simulink model "turbo_controller"  (R2025a)
settings: Solver=FixedStepAuto  StartTime=0.0  StopTime=inf  FixedStep=0.001  RelTol=1e-3
PostLoadFcn:
  | % 自动定位同目录CubeMX文件；不需要外部初始化脚本。
  | codertarget.data.setParameterValue('turbo_controller','STM32CubeMX.ProjectFile',fullfile(fileparts(get_param('turbo_controller','FileName')),'turbo_f407.ioc'));
InitFcn:
  | % 中文说明：按原控制器字段与类型创建三组接口总线；控制参数已内嵌。
  | tc_names=["EValve_Cycle" "EValve_Open" "Eblast_Cycle" "Eblast_Open" "Motor_Cycle" "Motor_Open" "EValve_Enable" "Eblast_Enable" "Motor_Enable" "SWO_Firework" "SWO_BleedAir" "EngineState" "Flag_ECUReset_Clear" "Flag_ECUReset_Save" "Flag_Reset_Enable" "Accelerator" "Nc_dem" "Nc"]; tc_types=["uint16" "uint16" "uint16" "uint16" "uint16" "uint16" "uint8" "uint8" "uint8" "uint8" "uint8" "uint8" "uint8" "uint8" "uint8" "single" "single" "single"];
  | for tc_k=1:numel(tc_names)
  |  tc_e(tc_k)=Simulink.BusElement; tc_e(tc_k).Name=char(tc_names(tc_k)); tc_e(tc_k).DataType=char(tc_types(tc_k));
  | end
  | EngineControl_Out=Simulink.Bus; EngineControl_Out.DataScope='Exported'; EngineControl_Out.Elements=tc_e;
  | clear tc_e tc_names tc_types tc_k
  | tc_names=["savedata1" "savedata2" "savedata3" "savedata4" "savedata5" "savedata6" "savedata7" "savedata8" "savedata9" "savedata10" "savedata11" "savedata12" "savedata13" "savedata14" "savedata15" "savedata16" "savedata17" "savedata18" "savedata19" "savedata20" "savedata21" "savedata22" "savedata23" "savedata24" "savedata25"]; tc_types=["single" "single" "single" "single" "single" "single" "single" "single" "single" "single" "single" "single" "single" "single" "single" "single" "single" "single" "single" "single" "single" "single" "single" "single" "single"];
  | for tc_k=1:numel(tc_names)
  |  tc_e(tc_k)=Simulink.BusElement; tc_e(tc_k).Name=char(tc_names(tc_k)); tc_e(tc_k).DataType=char(tc_types(tc_k));
  | end
  | SaveData_Out=Simulink.Bus; SaveData_Out.DataScope='Exported'; SaveData_Out.Elements=tc_e;
  | clear tc_e tc_names tc_types tc_k
  | tc_names=["senddata1" "senddata2" "senddata3" "senddata4" "senddata5" "senddata6" "senddata7" "senddata8" "senddata9" "senddata10" "senddata11" "senddata12" "senddata13" "senddata14" "senddata15" "senddata16" "senddata17" "senddata18" "senddata19" "senddata20" "senddata21" "senddata22" "senddata23" "senddata24" "senddata25" "senddata26" "senddata27" "senddata28" "senddata29"]; tc_types=["uint8" "uint8" "uint8" "uint8" "uint8" "uint8" "uint8" "uint8" "uint8" "uint8" "uint8" "uint8" "uint8" "uint8" "uint8" "uint8" "uint8" "uint8" "uint8" "uint8" "uint8" "uint8" "uint8" "uint8" "uint8" "uint8" "uint8" "uint8" "uint8"];
  | for tc_k=1:numel(tc_names)
  |  tc_e(tc_k)=Simulink.BusElement; tc_e(tc_k).Name=char(tc_names(tc_k)); tc_e(tc_k).DataType=char(tc_types(tc_k));
  | end
  | SendData_Out=Simulink.Bus; SendData_Out.DataScope='Exported'; SendData_Out.Elements=tc_e;
  | clear tc_e tc_names tc_types tc_k
  | 
  | % 以下为接口中文说明；只设置描述，不改变数值或数据类型。
  | EngineControl_Out.Description='执行控制输出（阀、电机、点火、状态及复位请求）';
  | tc_cn=["EValve_Cycle（主油阀周期计数（每计数2毫秒））" "EValve_Open（主油阀开通计数（每计数2毫秒））" "Eblast_Cycle（副油阀周期计数（每计数2毫秒））" "Eblast_Open（副油阀开通计数（每计数2毫秒））" "Motor_Cycle（起动电机周期计数）" "Motor_Open（起动电机开通计数）" "EValve_Enable（主油阀驱动使能）" "Eblast_Enable（副油阀驱动使能）" "Motor_Enable（起动电机使能）" "SWO_Firework（点火器使能（1开））" "SWO_BleedAir（引气阀使能（1开））" "EngineState（发动机状态）" "Flag_ECUReset_Clear（清除复位恢复状态请求）" "Flag_ECUReset_Save（保存复位恢复数据请求）" "Flag_Reset_Enable（处理器软件复位请求）" "Accelerator（油门／油泵给定控制量）" "Nc_dem（控制目标转速）" "Nc（发动机反馈转速（转每分））"];
  | tc_elements=EngineControl_Out.Elements;
  | for tc_k=1:numel(tc_cn)
  |  tc_elements(tc_k).Description=char(tc_cn(tc_k));
  | end
  | EngineControl_Out.Elements=tc_elements;
  | clear tc_cn tc_elements tc_k
  | SaveData_Out.Description='25项运行记录；字段含义按当前模型数据来源解释';
  | tc_cn=["savedata1（指令回显记录）" "savedata2（入口总温记录（℃））" "savedata3（电源电压记录）" "savedata4（排气温度记录（℃））" "savedata5（标定燃油压力记录）" "savedata6（副油阀占空比记录（％））" "savedata7（主油阀占空比记录（％））" "savedata8（温度修正转速记录）" "savedata9（开关输出及反馈位域）" "savedata10（物理转速记录）" "savedata11（油泵目标给定原始值）" "savedata12（起动电机占空比记录（％））" "savedata13（发动机状态码记录）" "savedata14（故障告警位域记录）" "savedata15（模型记录帧序号）" "savedata16（处理器温度记录（℃））" "savedata17（装订转速记录（沿用旧电源字段名））" "savedata18（导航高度记录）" "savedata19（飞行空速记录）" "savedata20（主阀旧记录位（恒零保留））" "savedata21（第21项保留记录（恒零））" "savedata22（保留记录项22）" "savedata23（保留记录项23）" "savedata24（保留记录项24）" "savedata25（保留记录项25）"];
  | tc_elements=SaveData_Out.Elements;
  | for tc_k=1:numel(tc_cn)
  |  tc_elements(tc_k).Description=char(tc_cn(tc_k));
  | end
  | SaveData_Out.Elements=tc_elements;
  | clear tc_cn tc_elements tc_k
  | SendData_Out.Description='29字段回传及外设命令接口；板端上位机帧只取第3至27字段';
  | tc_cn=["senddata1（回传发送允许标志（不直接上线路））" "senddata2（回传载荷长度25字节）" "senddata3（回传指令回显字节）" "senddata4（总温编码字节（℃＋80））" "senddata5（电源电压编码字节）" "senddata6（排温编码高字节）" "senddata7（排温编码低字节）" "senddata8（燃油压力编码高字节）" "senddata9（燃油压力编码低字节）" "senddata10（副油阀占空比字节（％））" "senddata11（主油阀占空比字节（％））" "senddata12（修正转速编码高字节）" "senddata13（修正转速编码低字节）" "senddata14（驱动及反馈状态位域）" "senddata15（物理转速编码高字节）" "senddata16（物理转速编码低字节）" "senddata17（油泵目标给定高字节（串口二使用））" "senddata18（油泵目标给定低字节（串口二使用））" "senddata19（起动电机占空比命令（串口一使用））" "senddata20（发动机状态码字节）" "senddata21（故障告警位域字节）" "senddata22（帧序号占位（板端另行填写））" "senddata23（处理器温度编码（℃＋50））" "senddata24（控制目标转速编码高字节）" "senddata25（控制目标转速编码低字节）" "senddata26（占位字节（板端改填实测泵速高字节））" "senddata27（占位字节（板端改填实测泵速低字节））" "senddata28（装订转速高字节（本板未发送））" "senddata29（装订转速低字节（本板未发送））"];
  | tc_elements=SendData_Out.Elements;
  | for tc_k=1:numel(tc_cn)
  |  tc_elements(tc_k).Description=char(tc_cn(tc_k));
  | end
  | SendData_Out.Elements=tc_elements;
  | clear tc_cn tc_elements tc_k
  | 
  | 
  | % FRAM模块化事务：接口类型和上电初始状态，随模型保存，无外部初始化文件。
  | clear FM_elements
  | FM_elements(1)=Simulink.BusElement;FM_elements(1).Name='phase';FM_elements(1).DataType='uint8';FM_elements(1).Dimensions=[1 1];FM_elements(1).Description='phase（当前事务阶段）';
  | FM_elements(2)=Simulink.BusElement;FM_elements(2).Name='a';FM_elements(2).DataType='uint8';FM_elements(2).Dimensions=[64 1];FM_elements(2).Description='a（启动时缓存的首区64字节）';
  | FM_elements(3)=Simulink.BusElement;FM_elements(3).Name='active';FM_elements(3).DataType='uint16';FM_elements(3).Dimensions=[1 1];FM_elements(3).Description='active（当前有效记录区地址）';
  | FM_elements(4)=Simulink.BusElement;FM_elements(4).Name='generation';FM_elements(4).DataType='uint32';FM_elements(4).Dimensions=[1 1];FM_elements(4).Description='generation（当前有效记录代号）';
  | FM_elements(5)=Simulink.BusElement;FM_elements(5).Name='record';FM_elements(5).DataType='uint8';FM_elements(5).Dimensions=[64 1];FM_elements(5).Description='record（本次冻结的待写记录）';
  | FM_elements(6)=Simulink.BusElement;FM_elements(6).Name='addr';FM_elements(6).DataType='uint16';FM_elements(6).Dimensions=[1 1];FM_elements(6).Description='addr（本次备用写入地址）';
  | FM_elements(7)=Simulink.BusElement;FM_elements(7).Name='lastSave';FM_elements(7).DataType='single';FM_elements(7).Dimensions=[1 1];FM_elements(7).Description='lastSave（上次开始保存的秒数）';
  | FM_elements(8)=Simulink.BusElement;FM_elements(8).Name='lastState';FM_elements(8).DataType='uint8';FM_elements(8).Dimensions=[1 1];FM_elements(8).Description='lastState（上次保存时的发动机状态）';
  | FM_elements(9)=Simulink.BusElement;FM_elements(9).Name='boot';FM_elements(9).DataType='boolean';FM_elements(9).Dimensions=[1 1];FM_elements(9).Description='boot（启动记录是否允许恢复）';
  | FM_elements(10)=Simulink.BusElement;FM_elements(10).Name='consumed';FM_elements(10).DataType='boolean';FM_elements(10).Dimensions=[1 1];FM_elements(10).Description='consumed（本次启动恢复通知是否已发送）';
  | FM_elements(11)=Simulink.BusElement;FM_elements(11).Name='payload';FM_elements(11).DataType='uint8';FM_elements(11).Dimensions=[20 1];FM_elements(11).Description='payload（当前20字节恢复内容）';
  | ... (+35 lines)
model workspace (MAT data in the model file):
  CRC16_Table_Reference = [0 4129 8258 12387 16516 20645 24774 28903 33032 37161 41290 45419 ... (256 elements, 256x1)]
  PE_Kaer = [0.15402 0.15402 0.12264 0.10076 0.09481 0.07601 0.07111 0.0569 0.05198 0.04926 0.05308 0.04325 ... (13 elements, 1x13)]
  PE_Nr = [21.2982 61.4260372 67.7475458 72.7394382 76.845934 80.6988798 83.8449282 86.6491912 88.9382406 89.178606 91.1938214 93.4068058 ... (13 elements, 1x13)]
  PE_Pump_Translate = 33.5999984741
  PE_RotaSpeed_Translate = 860
  PE_Taer = [0.4939154 0.4939154 0.40780982 0.34066978 0.31622756 0.30405716 0.34300244 0.26785022 0.37393554 0.23914836 0.44563948 0.31044662 ... (13 elements, 1x13)]
  PF_ACCFULLRANGE = 3360
  PF_Flag_ECUReset = 0
  PF_Flag_rx_suc = 1
  PF_Gear_Info = [40000; 45000; 50000; 55000; 57000; 59000; 60000; 61000; 61000; 61000; 61000; 61000]
  PF_K_TiaoJie = 1
  PF_Kpu = 10
  PF_MySet_Rxdata = [0 0 0 0 0 0 0 0 0 0 0 0 ... (50 elements, 50x1)]
  PF_MyUsart1_Rxdata = [0 0 0 0 0 0 0 0 0 0 0 0 ... (50 elements, 50x1)]
  PF_MyUsart2_Rxdata = [0 0 0 0 0 0 0 0 0 0 0 0 ... (50 elements, 50x1)]
  PF_Reset_Information = [0 0 0 0 0 0 0 0 0 0 0 0 ... (20 elements, 20x1)]
  PF_Sensor_X1_T4 = [0 4095]
  PF_Sensor_X2_T4 = [0 1.66666698456]
  PF_Sensor_X3_T4 = [0 504 999 1497 2010 2529 3051 3568 4076 4571 4959]
  PF_Sensor_X_P2 = [0.5 3]
  PF_Sensor_X_Poil = [0.5 3]
  PF_Sensor_X_T1t = [-50 300]
  PF_Sensor_X_Vpower = [0 3]
  PF_Sensor_X_Vpump = [0 3]
  PF_Sensor_Y1_T4 = [0 3]
  PF_Sensor_Y2_T4 = [0 5000]
  PF_Sensor_Y3_T4 = [0 100 200 300 400 500 600 700 800 900 980]
  PF_Sensor_Y_P2 = [0 1000]
  PF_Sensor_Y_Poil = [0 1000]
  PF_Sensor_Y_T1t = [-50 300]
  PF_Sensor_Y_Vpower = [0 33]
  PF_Sensor_Y_Vpump = [0 33]
  PG_CtrlMode_CloseLoop : mpt.Parameter (value not decoded)
  PG_CtrlMode_ManualAcc : mpt.Parameter (value not decoded)
  PG_CtrlMode_Origin : mpt.Parameter (value not decoded)
  PG_CtrlMode_Start : mpt.Parameter (value not decoded)
  PG_CtrlMode_Stop : mpt.Parameter (value not decoded)
  PG_ES_Clp : mpt.Parameter (value not decoded)
  PG_ES_EngStart : mpt.Parameter (value not decoded)
  PG_ES_Manual : mpt.Parameter (value not decoded)
  PG_ES_Origin : mpt.Parameter (value not decoded)
  PG_ES_Stop : mpt.Parameter (value not decoded)
  PG_Instr_BleedAirSet : mpt.Parameter (value not decoded)
  PG_Instr_CloseLoop : mpt.Parameter (value not decoded)
  PG_Instr_ECUReSet : mpt.Parameter (value not decoded)
  PG_Instr_EValveSet : mpt.Parameter (value not decoded)
  PG_Instr_EblastSet : mpt.Parameter (value not decoded)
  PG_Instr_Erase : mpt.Parameter (value not decoded)
  PG_Instr_FireWorkSet : mpt.Parameter (value not decoded)
  PG_Instr_ManualPlus : mpt.Parameter (value not decoded)
  PG_Instr_ManualrReduce : mpt.Parameter (value not decoded)
  PG_Instr_MotorSet : mpt.Parameter (value not decoded)
  PG_Instr_OilSet : mpt.Parameter (value not decoded)
  PG_Instr_SelfCheck : mpt.Parameter (value not decoded)
  PG_Instr_Start : mpt.Parameter (value not decoded)
  PG_Instr_Stop : mpt.Parameter (value not decoded)
  PG_Instr_StopZero : Simulink.Parameter (value not decoded)
  PG_Location_Air : Simulink.Parameter (value not decoded)
  PG_Location_Gnd : Simulink.Parameter (value not decoded)
  PG_ServoCtrlMode_CloseLoop : Simulink.Parameter (value not decoded)
  PG_ServoCtrlMode_CloseLoopMax : Simulink.Parameter (value not decoded)
  PG_ServoCtrlMode_CloseLoopMin : Simulink.Parameter (value not decoded)
  PG_ServoCtrlMode_ManualAcc : Simulink.Parameter (value not decoded)
  PG_ServoCtrlMode_ManualAccMax : Simulink.Parameter (value not decoded)
  PG_ServoCtrlMode_ManualAccMin : Simulink.Parameter (value not decoded)
  PG_SpeedDot_Permit : Simulink.Parameter (value not decoded)
  PL_EngineModel_Actuator = [0 10 100]
  PL_EngineModel_EngineStar_Press_P2 = [1013 1098.4 1099.144828 1099.931034 1103.613793 1162.662069 1143.793103 1131.006897 1123.186207 1117.6 1114 1111.806897 ... (127 elements, 1x127)]
  PL_EngineModel_EngineStar_RotaSpeed = [200 2000 9584 9660 10220 10240 10260 10288 10308 10368 10380 10408 ... (127 elements, 1x127)]
  PL_EngineModel_EngineStar_Temp_Exhaust = [128 129 129.1 130 131 131.1 132 133 134 134.1 135 135.1 ... (127 elements, 1x127)]
  PL_EngineModel_EngineStar_Time = [0.05 0.1 0.15 0.2 0.25 0.3 0.35 0.4 0.45 0.5 0.55 0.6 ... (127 elements, 1x127)]
  PL_EngineModel_IdleAbove_Nr = [0 21.2982 61.4260372 67.7475458 72.7394382 76.845934 80.6988798 83.8449282 86.6491912 88.9382406 89.178606 91.1938214 ... (14 elements, 1x14)]
  PL_EngineModel_IdleAbove_P2r = [0.986923266716 1.57907722675 1.81593881076 1.99358499877 2.23044658278 2.43770046879 2.65482358747 2.84233900814 3.03972366149 3.18776215149 3.25684678016 3.3950160375 ... (14 elements, 1x14)]
  PL_EngineModel_IdleAbove_Tempr = [0.0536001429337 1.07200285867 1.63301768805 1.63659103091 1.66875111667 1.72592460247 1.77595140254 1.86171163123 1.95461854565 2.03323208862 2.03323208862 2.13685903162 ... (14 elements, 1x14)]
  PL_EngineModel_IdleAbove_Ter = [0.42434128 0.42434128 0.42434128 0.30669408 0.23570008 0.22150128 0.1997974 0.23803274 0.16115638 0.24279948 0.13600422 0.31308354 ... (14 elements, 1x14)]
  PL_EngineModel_IdleAbove_Wfr = [0 10.142 23.8337 27.8905 31.9473 36.0041 40.0609 44.1177 48.1745 52.2313 52.7384 56.7952 ... (14 elements, 1x14)]
  PL_EngineModel_Press_P2 = [400 400 400 400 400 400 400 400 400 400]
  PL_EngineModel_Rotaspeed = [0 20000 96400]
  PL_EngineModel_Temp_Exhaust = [500 500 500 500 500 500 500 500 500 500]
  PL_Kaer = [0.1 0.1 0.1 0.1 0.1 0.1]
  PL_Nr = [50 60 70 80 90 100]
  PL_Taer = [0.1 0.1 0.1 0.1 0.1 0.1]
  Sig : Simulink.Signal (value not decoded)
  Ts_ms : Simulink.Parameter (value not decoded)
  false : Simulink.Parameter (value not decoded)
  true : Simulink.Parameter (value not decoded)
symbols that are objects in the model workspace (value not decoded): PG_CtrlMode_CloseLoop, PG_CtrlMode_ManualAcc, PG_CtrlMode_Origin, PG_CtrlMode_Start, PG_CtrlMode_Stop, PG_ES_Clp, PG_ES_EngStart, PG_ES_Manual, PG_ES_Origin, PG_ES_Stop, PG_Instr_BleedAirSet, PG_Instr_CloseLoop, PG_Instr_EblastSet, PG_Instr_ECUReSet, PG_Instr_Erase, PG_Instr_EValveSet, PG_Instr_FireWorkSet, PG_Instr_ManualPlus, PG_Instr_ManualrReduce, PG_Instr_MotorSet, PG_Instr_OilSet, PG_Instr_SelfCheck, PG_Instr_Start, PG_Instr_Stop, PG_Instr_StopZero, PG_ServoCtrlMode_CloseLoop, PG_ServoCtrlMode_CloseLoopMax, PG_ServoCtrlMode_CloseLoopMin, PG_ServoCtrlMode_ManualAcc, PG_ServoCtrlMode_ManualAccMax, PG_ServoCtrlMode_ManualAccMin, Ts_ms
libraries: simulink x97, stm32blockslib x10, stm32f4xxblockslib x8
(part 7 of 26)

== system turbo_controller/BoardInput_输入换算与协议解析/In03_Pump（油泵回包预留校验） ==
  note: 输入侧油泵回包的预留检查
      |
      | 本模块接收油泵串口字节和有效数量，内部Receive按AA55帧头拼接22字节帧，再检查CRC16。分批到达
      | 的帧可以依靠缓存接着收，校验失败不会变成有效帧。
      |
      | 它保留的是输入侧原有预留校验路径，当前该结果没有用来更新控制转速或实际回传泵速。不要因为这
      | 里名为Pump，就把它当成最终泵速反馈来源。
      |
      | 实际用于上位机回传的油泵反馈，在BoardOutput/Out01_Pump中处理：同样检查22字节帧，提取第6、7
      | 字节并作0.875/0.125平滑。本模块没有取代那条路径，也不生成发往油泵的控制命令。
  Rx（串口接收字节）_237 : Inport  OutDataTypeStr=uint8
  Count（有效字节数）_238 : Inport  Port=2  OutDataTypeStr=uint32
  Format（保持原输出维度）_1 : Reshape
  Receive（逐字节组帧与保持有效结果）_353 : Subsystem  Description=|
      | 预留油泵校验接收流程：按1→2→3→4阅读
      | 
      | 第一步只遍历本批有效字节，最多处理64项；第二步识别AA55、收齐22字节，并保存尚未收完的半帧；第三步确认本字节刚收齐且CRC通过；第四步统计这一批是否出现过有效帧。
      | 
      | Loop在一次调用内逐字节重复这些步骤，不是每一步各等1 ms。接收数组的Index每批重新遍历，收帧Position可以跨批保留，两者不是同一个位置。
      | 
      | 本分支输出本批是否出现有效帧，不生成实际平滑泵速。实际泵速来自BoardOutput/Out01_Pump的接收路径。
      | 
      | 本次将原有处理块按职责封装，保留原协议、初始化、数据类型、校验和循环行为。各步骤内部可看输入、公式和例子。
  Valid（原预留校验结果）_354 : Outport
  wires:
  Rx（串口接收字节）_237/1 -> Receive（逐字节组帧与保持有效结果）_353/1(Rx（本次接收字节）_239)  "Rx（串口接收字节）"
  Count（有效字节数）_238/1 -> Receive（逐字节组帧与保持有效结果）_353/2(Count（本次有效字节数）_240)  "Count（有效字节数）"
  Receive（逐字节组帧与保持有效结果）_353/1(Valid（原预留校验结果）_352) -> Format（保持原输出维度）_1/1  "Receive（逐字节组帧与保持有效结果）"
  Format（保持原输出维度）_1/1 -> Valid（原预留校验结果）_354/1

== system turbo_controller/BoardInput_输入换算与协议解析/In04_Capture（捕获间隔缓存） ==
  note: 捕获间隔缓存：把脉冲发生时刻整理成最近十个时间间隔
      |
      | 输入Capture是TIM3本批捕获读数，最多16项；输入Count只说明本批有几项新读数，Seconds为本次处
      | 理时刻，单位秒。当前定时器每增加1计数相当于1微秒。
      |
      | 按四块阅读：
      | Step01逐项取出本批有效捕获，超过本批数量或第16项就结束循环；
      | Step02保存上次捕获、十项间隔、写入位置、累计有效数和最近有效时间；
      | Step03根据本项捕获计算间隔，决定是否更新缓存和状态；
      | Step04只整理三个输出的维度，送后续测速。
      |
      | Step02与Step03之间是状态反馈，不是先等一个额外毫秒再处理。Loop会在同一次调用内遍历本批多个
      | 捕获；一个批次的末项读数也会留作下一批首项的差分基准。
      |
      | 输出Periods为最近十个间隔，Count为缓存里真正有效的间隔个数，LastTime为最近接受正间隔的处理
      | 时刻。输出Count与输入Count不是同一个数量。这里不直接输出转速；去极值与每转3脉冲换算在In05_
      | Speed/CaptureSpeed完成。
  Capture（最多十六个捕获计数）_355 : Inport  OutDataTypeStr=uint16
  Count（本次有效个数）_356 : Inport  Port=2  OutDataTypeStr=uint32
  Seconds（当前秒数）_357 : Inport  Port=3  OutDataTypeStr=double
  Loop（逐项处理循环）_358 : ForIterator  IterationLimit=16  ExternalIncrement=on  IterationVariableDataType=uint32
  Step01_逐项取出本批有效捕获 : Subsystem  Description=|
      | 第一步：按顺序取出本批捕获，不处理数组尾部旧值
      | 
      | 外层Loop给出从1开始的序号i。本项捕获=Capture(i)，本项有效=(i≤本批Count)。
      | 
      | 如果i已达到本批Count，或i=16，就把下一循环序号设17，结束循环；否则下一序号=i+1。因此输入数组虽然有16项，Count=3时只会把前3项当新捕获。Count=0时保留一次无效项处理，状态由后面保持，不写入新间隔。
      | 
      | 例：一批有[1000,2000,3000]三项，依次交给更新步骤处理；它们是在本次调用内顺序处理，不是分三毫秒执行。
      | 
      | 输出分别为本项捕获、有效许可和下一循环序号。i是本批数组位置，不是十项环形缓存的写入位置。
  Step02_保存捕获与缓存历史状态 : Subsystem  Description=|
      | 第二步：保留下一项计算还要用到的五种历史状态
      | 
      | 这里的五条记忆各有用途：
      | Previous：上一项有效捕获读数，用来求下一次差分，初值0；
      | Ring：最近十个已接受间隔，初值为十个0；
      | Index：下一次覆盖缓存的哪一项，初值1；
      | Count：已保存多少个有效间隔，初值0，最多10；
      | LastTime：最近接受正间隔的处理时刻，初值-1秒。
      | 
      | 每次把Step03给出的新状态按原类型保存：Previous为uint32，Index和Count为uint8，Ring和LastTime为single；下一次循环/调用再提供给Step03。
      | 
      | 不要把Previous、Ring和LastTime混为一份数据。读数用于差分，间隔用于测速，时间用于判断新鲜程度。没有有效捕获时，上游选择器会把旧状态送回来，记忆继续保持。
  Step03_计算间隔并更新环形缓存 : Subsystem  Description=|
      | 对一项捕获完成回卷差分和缓存更新
      | 
      | 输入为上一捕获、旧十项缓存、旧写入位置、旧有效数、旧最近时间，以及本次Capture、Seconds和Active。
      | 
      | 六步各做一件事：算回卷后的间隔、判断能否接受、生成缓存候选值、计算下一写入位置、计算有效数量、最后按许可提交状态。
      | 
      | 关键规则有两条：只要Active为真就更新Previous；但只有Active为真且间隔>0，才更新Ring、Index、Count和LastTime。重复读数的零间隔不会增加记录，也不刷新最近有效时间。
      | 
      | 例：上次65530、这次4，间隔为10；若本项有效，就存10并更新状态。若本项无效，即使算出了10，也保留全部旧状态。输出回到In04的历史记忆供下一项使用，不是给硬件发送命令。
  Step04_整理间隔数量和时间输出 : Subsystem  Description=|
      | 第四步：整理三个对外输出的形状，不再次计算
      | 
      | 将Step03输出的十项Ring整理为原工程的一维向量接口；累计有效数量和最近有效时间按原来要求整理为标量形状。
      | 
      | 数值不变、单位不变，也不做新的滤波。Periods仍是计数间隔，当前配置下可按微秒解释；Count仍为0～10；LastTime仍为秒。
      | 
      | 例如Ring中一项1000经过此处还是1000，不会变成1000转/分。真正的转速换算在后面的CaptureSpeed，超时判断在Status；本块只保证连接双方看到的数组形状与修改前一致。
  Periods（最近十个有效间隔）_416 : Outport
  Count（有效间隔数）_417 : Outport  Port=2
  LastTime（最近有效脉冲秒数）_418 : Outport  Port=3
  wires:
  Step04_整理间隔数量和时间输出/3(输出3_Format（保持原输出维度）) -> LastTime（最近有效脉冲秒数）_418/1
  Step04_整理间隔数量和时间输出/2(输出2_Format（保持原输出维度）) -> Count（有效间隔数）_417/1
  Step04_整理间隔数量和时间输出/1(输出1_Vector1D（保持原一维向量接口）) -> Periods（最近十个有效间隔）_416/1
  Step01_逐项取出本批有效捕获/3(输出3_本项捕获有效) -> Step03_计算间隔并更新环形缓存/8(Active（本项捕获有效）_381)
  Step01_逐项取出本批有效捕获/2(输出2_本项捕获读数) -> Step03_计算间隔并更新环形缓存/6(Capture（当前捕获计数）_379)
  Step02_保存捕获与缓存历史状态/5(输出5_上次有效间隔时刻) -> Step03_计算间隔并更新环形缓存/5(LastTime（最近有效脉冲时间）_378)
  Step02_保存捕获与缓存历史状态/4(输出4_累计有效间隔数) -> Step03_计算间隔并更新环形缓存/4(Count（有效间隔个数）_377)
  Step02_保存捕获与缓存历史状态/3(输出3_当前环形写入位置) -> Step03_计算间隔并更新环形缓存/3(Index（下一写入位置）_376)
  Step02_保存捕获与缓存历史状态/2(输出2_旧十项间隔缓存) -> Step03_计算间隔并更新环形缓存/2(Ring（十项间隔缓存）_375)
  Step02_保存捕获与缓存历史状态/1(输出1_上一捕获读数) -> Step03_计算间隔并更新环形缓存/1(Previous（上次捕获计数）_374)
  Step01_逐项取出本批有效捕获/1(输出1_下一序号或退出值17) -> Loop（逐项处理循环）_358/1
  Step03_计算间隔并更新环形缓存/4(Count（更新后的有效个数）_411) -> Step04_整理间隔数量和时间输出/1(输入1_更新后的有效间隔数), Step02_保存捕获与缓存历史状态/5(输入5_更新后的有效间隔数)  "更新后的有效间隔数"
  Step03_计算间隔并更新环形缓存/3(Index（下次写入位置）_409) -> Step02_保存捕获与缓存历史状态/4(输入4_下一环形写入位置)  "下一环形写入位置"
  Step03_计算间隔并更新环形缓存/1(Previous（下次差分基准）_405) -> Step02_保存捕获与缓存历史状态/3(输入3_下一差分基准)  "下一差分基准"
  Step03_计算间隔并更新环形缓存/5(LastTime（最近有效脉冲时间）_414) -> Step02_保存捕获与缓存历史状态/2(输入2_最近有效间隔处理时刻), Step04_整理间隔数量和时间输出/2(输入2_最近有效间隔处理时刻)  "最近有效间隔处理时刻"
  Step03_计算间隔并更新环形缓存/2(Ring（更新后的间隔缓存）_407) -> Step04_整理间隔数量和时间输出/3(输入3_更新后的十项间隔), Step02_保存捕获与缓存历史状态/1(输入1_更新后的十项间隔)  "更新后的十项间隔"
  Capture（最多十六个捕获计数）_355/1 -> Step01_逐项取出本批有效捕获/3(输入3_本批最多16项捕获数组)  "本批最多16项捕获数组"
  Count（本次有效个数）_356/1 -> Step01_逐项取出本批有效捕获/2(输入2_本批有效捕获个数)  "本批有效捕获个数"
  Loop（逐项处理循环）_358/1 -> Step01_逐项取出本批有效捕获/1(输入1_本批当前处理序号)  "本批当前处理序号"
  Seconds（当前秒数）_357/1 -> Step03_计算间隔并更新环形缓存/7(Seconds（当前秒数）_380)  "Seconds（当前秒数）"

== system turbo_controller/BoardInput_输入换算与协议解析/In05_Speed（转速来源选择与滤波） ==
  note: 电机反馈与捕获估速怎样选成控制转速
      |
      | 这里有两种候选转速：电机串口反馈Motor，以及十项捕获间隔算出的Captured。输出Speed送根层Cont
      | rolRate，再到ISM作进一步异常判断和滤波。
      |
      | 先由Clock20ms产生每20 ms更新许可。CaptureSpeed从有效间隔中去掉一个最大和一个最小，估算转速
      | ，并给出分母有效标志。Status判断：上一电机给定是否非零、是否还在10次节拍等待中、脉冲是否超
      | 过0.1 s未更新、间隔是否至少3项。
      |
      | Select按顺序选择：电机给定非零时优先Motor，并把等待计数清零；退出电机后先保持旧Speed，等待
      | 10次20 ms节拍，约0.2 s后再尝试捕获估速。
      | 等待结束后，脉冲超时则给零；未超时且数量足够、分母有效才采用Captured，否则保持旧值。
      |
      | 非20 ms更新时刻，Speed和等待计数都保持。因此“父级每1 ms运行”并不是每1 ms都切换转速来源。
      | Held是上次控制转速，WaitCount是切换过程的记忆。
  Periods（最近十项捕获间隔）_1 : Inport  OutDataTypeStr=single
  Count（有效间隔数）_2 : Inport  Port=2  OutDataTypeStr=uint8
  LastTime（最近脉冲时间）_3 : Inport  Port=3  OutDataTypeStr=single
  PreviousMotor（上一电机给定）_4 : Inport  Port=4  OutDataTypeStr=uint16
  MotorSpeed（电机反馈转速）_5 : Inport  Port=5  OutDataTypeStr=single
  Seconds（当前秒数）_6 : Inport  Port=6  OutDataTypeStr=double
  CaptureSpeed（去极值估算转速）_19 : Subsystem  Description=|
      | 把最近脉冲间隔换算成转速：先筛数据，再去极值，最后计算
      | 
      | 输入Periods最多十项，Count=n说明前几项有效。四步分别是：排除空位、去掉一个最大值和一个最小值、检查分母并避免除零、按每转3脉冲换算RPM。
      | 
      | 去极值后的和S=有效间隔之和-最大有效间隔-最小有效间隔。
      | 转速=60000000×(n-2)/(3×S)，间隔采用微秒时，输出单位为转/分。
      | 
      | 例如十项都为1000微秒，去掉两项后S=8000，转速=60000000×8/(3×8000)=20000。去极值减轻单个偏大/偏小间隔的影响，不是无条件识别所有错误脉冲。
      | 
      | 本模块Valid只表示S>0。至少有3项的要求、最近脉冲是否超时、是否优先采用电机串口反馈，由外层Status和Select决定。数据不足时即使这里有一个数，也不能绕过这些条件直接用作控制反馈。
  Clock20ms（二十毫秒更新节拍）_18 : Subsystem  Description=|
      | 从秒数产生每二十毫秒一次的许可
      | 
      | 本模块收到当前模型时间Seconds。先乘1000换成毫秒，再对20取余，判断余数是否小于1：
      | 工作许可 = mod(Seconds×1000,20)<1。
      | 
      | 在父级1 ms离散调用下，约在0、20、40、60 ms等时刻为真，中间毫秒为假。用“小于1”表示当前1 ms时间格，避免把它理解成连续时间的一次精确相等判断。
      | 
      | 这只是一个布尔许可，不会让模型等待或暂停。转速选择用它决定何时更新Speed，回传组帧用它决定何时生成新帧；其他1 ms任务继续正常运行。
  Format（保持原输出维度）_1 : Reshape
  Held（保持的控制转速）_7 : UnitDelay  InitialCondition=single(0)  SampleTime=-1  HasFrameUpgradeWarning=on
  Select（优先级与保持选择）_65 : Subsystem  Description=|
      | 按优先级决定这一周期输出哪种转速
      | 
      | 输入包含20 ms许可、四个来源条件、捕获分母有效标志，两种候选转速，以及上次Speed和等待次数。处理顺序很重要。
      | 
      | 先看20 ms许可：本毫秒不到更新时间，就保持上次Speed和等待次数。
      | 到更新时间后，如果UseMotor成立，直接采用电机反馈Motor，同时等待次数清零。
      | 如果不再使用Motor，但Waiting仍成立，则保持旧Speed，并将等待次数加1，最多等待10次节拍。
      | 
      | 等待结束后，先看捕获是否Timeout：超时就输出0。未超时时，Enough和Valid同时成立才采用Captured；数量不够或分母无效时仍保持Held。
      | 
      | 例如电机刚停止给定，不会立刻切到可能还未准备好的捕获值，而先保持约0.2 s。Speed和WaitCount输出在父级被保存，下一次再作为历史输入，所以不能删除这两条记忆反馈。
  Status（来源与超时判定）_39 : Subsystem  Description=|
      | 转速来源现在是否可用
      | 
      | 这里不计算转速，而把输入整理成四个供Select使用的布尔条件。
      | 
      | UseMotor：上一周期电机给定大于0，表示电机仍在被驱动，优先采用电机串口反馈。
      | Waiting：等待次数小于10，表示从电机反馈退出后还在过渡期。等待次数由外层按20 ms节拍推进，10次约0.2 s。
      | Timeout：当前秒数减最近有效脉冲时间大于0.1 s，表示捕获结果已经不够新鲜。
      | Enough：有效间隔数至少3，保证去掉最大和最小之后还有数据。
      | 
      | 例如已有10项间隔，但最后一次脉冲是0.3 s前，Enough虽为真，Timeout也为真，仍不能把旧估速当作当前转速。四个条件各表达一件事，由后面的Select按优先级合成决定。
  StoreSpeed（保存控制转速）_66 : DataTypeConversion  OutDataTypeStr=single  RndMeth=Round
  StoreWait（保存等待次数）_67 : DataTypeConversion  OutDataTypeStr=uint8  RndMeth=Round
  WaitCount（切换等待次数）_8 : UnitDelay  InitialCondition=uint8(0)  SampleTime=-1  HasFrameUpgradeWarning=on
  Speed（提供给控制模型的转速）_68 : Outport
  wires:
  [SP_Count] -> Status（来源与超时判定）_39/2(Count（有效间隔数）_21)  "SP_Count（有效间隔数）"
  PreviousMotor（上一电机给定）_4/1 -> Status（来源与超时判定）_39/1(PreviousMotor（上一电机给定）_20)  "PreviousMotor（上一电机给定）"
  [SP_Time] -> Clock20ms（二十毫秒更新节拍）_18/1(Seconds（当前秒数）_9)  "SP_Time（当前秒数）"
  CaptureSpeed（去极值估算转速）_19/1(Speed（定时器估算转速）_471) -> [SP_Capture]  "SP_Capture（捕获估算转速）"
  Periods（最近十项捕获间隔）_1/1 -> CaptureSpeed（去极值估算转速）_19/1(Periods（最近十项间隔）_444)  "Periods（最近十项捕获间隔）"
  MotorSpeed（电机反馈转速）_5/1 -> Select（优先级与保持选择）_65/7(Motor（电机反馈转速）_46)  "MotorSpeed（电机反馈转速）"
  [SP_Count] -> CaptureSpeed（去极值估算转速）_19/2(Count（有效项数）_445)  "SP_Count（有效间隔数）"
  [SP_Held] -> Select（优先级与保持选择）_65/9(Held（上次控制转速）_48)  "SP_Held（保持的控制转速）"
  Seconds（当前秒数）_6/1 -> [SP_Time]  "SP_Time（当前秒数）"
  [SP_Time] -> Status（来源与超时判定）_39/4(Seconds（当前秒数）_23)  "SP_Time（当前秒数）"
  [SP_Capture] -> Select（优先级与保持选择）_65/8(Captured（捕获估算转速）_47)  "SP_Capture（捕获估算转速）"
  LastTime（最近脉冲时间）_3/1 -> Status（来源与超时判定）_39/3(LastTime（最近脉冲秒数）_22)  "LastTime（最近脉冲时间）"
  [SP_Wait] -> Status（来源与超时判定）_39/5(WaitCount（切换等待次数）_24)  "SP_Wait（切换等待次数）"
  Count（有效间隔数）_2/1 -> [SP_Count]  "SP_Count（有效间隔数）"
  CaptureSpeed（去极值估算转速）_19/2(Valid（估算分母有效）_472) -> [SP_Valid]  "SP_Valid（估算分母有效）"
  [SP_Valid] -> Select（优先级与保持选择）_65/6(Valid（估算分母有效）_45)  "SP_Valid（估算分母有效）"
  Clock20ms（二十毫秒更新节拍）_18/1(Every20ms（二十毫秒更新许可）_17) -> Select（优先级与保持选择）_65/1(Control（二十毫秒许可）_40)  "Clock20ms（二十毫秒更新节拍）"
  Status（来源与超时判定）_39/1(UseMotor（电机反馈优先）_27) -> Select（优先级与保持选择）_65/2(UseMotor（电机反馈优先）_41)  "Status（来源与超时判定）"
  WaitCount（切换等待次数）_8/1 -> [SP_Wait]  "SP_Wait（切换等待次数）"
  Status（来源与超时判定）_39/2(Waiting（切换等待尚未完成）_30) -> Select（优先级与保持选择）_65/3(Waiting（切换等待中）_42)  "Status（来源与超时判定）"
  Status（来源与超时判定）_39/3(Timeout（捕获脉冲超时）_35) -> Select（优先级与保持选择）_65/4(Timeout（脉冲已超时）_43)  "Status（来源与超时判定）"
  Status（来源与超时判定）_39/4(Enough（有效间隔至少三个）_38) -> Select（优先级与保持选择）_65/5(Enough（间隔数足够）_44)  "Status（来源与超时判定）"
  [SP_Wait] -> Select（优先级与保持选择）_65/10(WaitCount（上次等待次数）_49)  "SP_Wait（切换等待次数）"
  Select（优先级与保持选择）_65/1(Speed（本次控制转速）_63) -> StoreSpeed（保存控制转速）_66/1, Format（保持原输出维度）_1/1  "Select（优先级与保持选择）"
  Select（优先级与保持选择）_65/2(WaitCount（下次等待次数）_64) -> StoreWait（保存等待次数）_67/1  "Select（优先级与保持选择）"
  Format（保持原输出维度）_1/1 -> Speed（提供给控制模型的转速）_68/1
  StoreSpeed（保存控制转速）_66/1 -> Held（保持的控制转速）_7/1  "StoreSpeed（保存控制转速）"
  StoreWait（保存等待次数）_67/1 -> WaitCount（切换等待次数）_8/1  "StoreWait（保存等待次数）"
  Held（保持的控制转速）_7/1 -> [SP_Held]  "SP_Held（保持的控制转速）"

== system turbo_controller/BoardInput_输入换算与协议解析/In06_Analog（模拟量换算） ==
  note: 八路ADC怎样变成五类测量数据
      |
      | 这里收到的是ADC1每20毫秒采集的一组八项计数，数值约为0～4095。计数表示输入电压在量程中的位
      | 置，还不能直接当成摄氏度或油压。本层先按数组位置分开处理，再把五类结果交给根层ControlRate
      | ，进入COMMRead_ISM/ISM继续标定。
      |
      | 1 电源电压取第1项。先转成single以便做小数运算，再计算：
      | 电源电压 = 第1项计数 × 48 / 4096，单位V。
      | 例如计数2048对应24 V。这里已完成电源电压换算，ISM随后直接把它放入Sensor.Vpower，用于22 V欠
      | 压判断、记录和回传。
      |
      | 2 控制器温度取第3项。这是芯片内部温度传感器的计数。本层只转成single后输出TECU；下一级Calib
      | rating_Tecu才把它换成电压和摄氏温度。本层没有把它当成温度直接使用。
      |
      | 3 排温取第4项，油压取第8项。两路在这里均只转成single，分别输出T4和POil。后面的Calibrating_
      | T4用三级查表得到排温，Calibrating_Poil用两级查表得到油压，然后各自低通滤波。它们离开本层时
      | 仍是ADC计数。
      |
      | 4 总温需要第5和第7两项一起计算。第5项提供参考电压，第7项提供传感器电压；TotalTemperature先
      | 反算电阻，再换算温度，最后加80形成T0编码。例如计算温度25 ℃时，编码为105；后面的Calibratin
      | g_T0再减80。
      |
      | 5 第2、第6项当前没有取出参与运算。Format/Reshape只整理输出的数组形状，不改变数值；single转
      | 换也不是物理标定。
      |
      | 因此，五个输出不能按同一种单位解释：Power是V，T4/TECU/POil仍是计数，T0是带80偏置的温度编码
      | 。这里的“数组第1项”对应硬件ADC通道2，并不是硬件通道1。
  ADC（八路原始采样）_69 : Inport  OutDataTypeStr=uint16
  Cast（数据类型转换）_{71,74,79,82} (4 alike) : DataTypeConversion  OutDataTypeStr=single  RndMeth=Round
  Constant（常量）_75 : Constant  Value=48/4096  OutDataTypeStr=single
  Format（保持原输出维度）_{1..5} (5 alike) : Reshape
  POil（第八路油压）_81 : Selector  InputPortWidth=8  IndexOptions=Index vector (dialog)  Indices=8  OutputSizes=1
  Power（第一路电源）_73 : Selector  InputPortWidth=8  IndexOptions=Index vector (dialog)  Indices=1  OutputSizes=1
  T4（第四路排温）_70 : Selector  InputPortWidth=8  IndexOptions=Index vector (dialog)  Indices=4  OutputSizes=1
  TECU（第三路处理器温度）_78 : Selector  InputPortWidth=8  IndexOptions=Index vector (dialog)  Indices=3  OutputSizes=1
  TotalTemperature（总温电阻与编码换算）_112 : Subsystem  Description=|
      | 两路电压怎样反算总温
      | 
      | 本模块位于In06_Analog内部，输入仍是完整八项ADC数组，但只用第5和第7项。第5项是测量电路的参考计数，第7项是温度传感器计数。计算的思路是先恢复电压，再由电路关系求电阻，最后由电阻标定得到温度。
      | 
      | 1 按现有电路比例恢复电压：
      | 参考电压 Vref = 第5项 × 3/4096 × 6/3.3；
      | 传感器电压 Vs = 第7项 × 3/4096；
      | 电压差 ΔV = Vref - Vs，以上单位均为V。
      | 这里的6/3.3是参考支路采用的比例，不能省略。
      | 
      | 2 当ΔV大于0.1 V时，采用有效电阻：
      | R = 1000 × Vs / ΔV。
      | 1000来自当前电路换算系数。例子：Vs为1 V、ΔV为1 V时，计算电阻为1000。
      | 
      | 3 将电阻换成温度：
      | 原始温度 = 0.25506 × R - 254.987696，单位℃；
      | 输出T0编码 = 原始温度 + 80。
      | 所以输出不是直接摄氏温度。后面ISM/Calibrating_T0会减80，并限制在-70～175 ℃。
      | 
      | 4 若ΔV不大于0.1 V，模型不采用这次除法结果，而输出替代电阻9999；分母选择支路也提供安全值，避免无效路径除零。该替代值继续换算后，会在下一级被限到175 ℃。这条处理没有另外输出“断线告警”，不能把175 ℃误认为一定是实测温度。
      | 
      | 本模块结果经In06_Analog和ControlRate16送入ISM。之后总温用于记录、回传及HuanSuanN温度修正转速；它没有直接接入Dynamic_Cal的参考温度输入。
  Voltage（电源电压换算）_76 : Product  Inputs=**  SaturateOnIntegerOverflow=on  OutDataTypeStr=Inherit: Same as first input
  T4（第四路排温计数）_72 : Outport
  Power（电源电压）_77 : Outport  Port=2
  TECU（第三路处理器温度计数）_80 : Outport  Port=3
  POil（第八路油压计数）_83 : Outport  Port=4
  T0（总温编码）_113 : Outport  Port=5
  wires:
  Constant（常量）_75/1 -> Voltage（电源电压换算）_76/2  "Constant（常量）"
  Cast（数据类型转换）_74/1 -> Voltage（电源电压换算）_76/1  "Cast（数据类型转换）"
  Power（第一路电源）_73/1 -> Cast（数据类型转换）_74/1  "Power（第一路电源）"
  ADC（八路原始采样）_69/1 -> T4（第四路排温）_70/1, POil（第八路油压）_81/1, Power（第一路电源）_73/1, TotalTemperature（总温电阻与编码换算）_112/1(ADC（八路原始采样）_84), TECU（第三路处理器温度）_78/1  "ADC（八路原始采样）"
  Format（保持原输出维度）_5/1 -> T0（总温编码）_113/1
  Format（保持原输出维度）_4/1 -> POil（第八路油压计数）_83/1
  Format（保持原输出维度）_3/1 -> TECU（第三路处理器温度计数）_80/1
  Format（保持原输出维度）_2/1 -> Power（电源电压）_77/1
  Format（保持原输出维度）_1/1 -> T4（第四路排温计数）_72/1
  T4（第四路排温）_70/1 -> Cast（数据类型转换）_71/1  "T4（第四路排温）"
  Cast（数据类型转换）_71/1 -> Format（保持原输出维度）_1/1  "Cast（数据类型转换）"
  Voltage（电源电压换算）_76/1 -> Format（保持原输出维度）_2/1  "Voltage（电源电压换算）"
  TECU（第三路处理器温度）_78/1 -> Cast（数据类型转换）_79/1  "TECU（第三路处理器温度）"
  Cast（数据类型转换）_79/1 -> Format（保持原输出维度）_3/1  "Cast（数据类型转换）"
  POil（第八路油压）_81/1 -> Cast（数据类型转换）_82/1  "POil（第八路油压）"
  Cast（数据类型转换）_82/1 -> Format（保持原输出维度）_4/1  "Cast（数据类型转换）"
  TotalTemperature（总温电阻与编码换算）_112/1(T0（总温编码）_111) -> Format（保持原输出维度）_5/1  "TotalTemperature（总温电阻与编码换算）"

== system turbo_controller/BoardInput_输入换算与协议解析/In07_GPIO（数字反馈映射） ==
  note: 把五路硬件电平解释成控制反馈
      |
      | 输入GPIOE按根层顺序包含PE13、PE14、PE15；GPIOD包含PD8、PD9。Selector按数组位置取出，再经过
      | 原有极性映射、single转换和形状整理，形成Fire、Main、Aux、Valve、Bleed五个输出。
      |
      | E口三项分别提供主阀、副阀、引气阀相关反馈；D口两项提供点火与阀使能/告警相关反馈。逻辑有效
      | 方向要结合本页取反支路：硬件低电平不一定表示软件“无告警”，因此不能把原始0/1直接当动作状
      | 态。
      |
      | 本层只整理反馈，不生成阀门驱动。输出经ControlRate进入ISM，按SWI_Firework、SWI_EValve等名称
      | 进入Sensor总线，供记录回传和有关检查使用。Format/Reshape只调整形状，类型转换不改变电路有效
      | 极性。
  GPIOE（E口三路输入）_530 : Inport  OutDataTypeStr=boolean
  GPIOD（D口两路输入）_531 : Inport  Port=2  OutDataTypeStr=boolean
  Aux（副阀反馈）_538 : Selector  InputPortWidth=3  IndexOptions=Index vector (dialog)  Indices=3  OutputSizes=1
  Bleed（放气反馈）_544 : Selector  InputPortWidth=3  IndexOptions=Index vector (dialog)  Indices=1  OutputSizes=1
  Cast（数据类型转换）_{533,536,539,542,545} (5 alike) : DataTypeConversion  OutDataTypeStr=uint8  RndMeth=Round
  Fire（点火反馈）_532 : Selector  InputPortWidth=2  IndexOptions=Index vector (dialog)  Indices=2  OutputSizes=1
  Format（保持原输出维度）_{1..5} (5 alike) : Reshape
  Main（主阀反馈）_535 : Selector  InputPortWidth=3  IndexOptions=Index vector (dialog)  Indices=2  OutputSizes=1
  Valve（阀使能反馈）_541 : Selector  InputPortWidth=2  IndexOptions=Index vector (dialog)  Indices=1  OutputSizes=1
  Fire（点火反馈）_534 : Outport
  Main（主阀反馈）_537 : Outport  Port=2
  Aux（副阀反馈）_540 : Outport  Port=3
  Valve（阀使能反馈）_543 : Outport  Port=4
  Bleed（放气反馈）_546 : Outport  Port=5
  wires:
  Fire（点火反馈）_532/1 -> Cast（数据类型转换）_533/1  "Fire（点火反馈）"
  GPIOD（D口两路输入）_531/1 -> Valve（阀使能反馈）_541/1, Fire（点火反馈）_532/1  "GPIOD（D口两路输入）"
  Bleed（放气反馈）_544/1 -> Cast（数据类型转换）_545/1  "Bleed（放气反馈）"
  GPIOE（E口三路输入）_530/1 -> Main（主阀反馈）_535/1, Aux（副阀反馈）_538/1, Bleed（放气反馈）_544/1  "GPIOE（E口三路输入）"
  Format（保持原输出维度）_1/1 -> Fire（点火反馈）_534/1
  Aux（副阀反馈）_538/1 -> Cast（数据类型转换）_539/1  "Aux（副阀反馈）"
  Cast（数据类型转换）_545/1 -> Format（保持原输出维度）_5/1  "Cast（数据类型转换）"
  Valve（阀使能反馈）_541/1 -> Cast（数据类型转换）_542/1  "Valve（阀使能反馈）"
  Main（主阀反馈）_535/1 -> Cast（数据类型转换）_536/1  "Main（主阀反馈）"
  Cast（数据类型转换）_533/1 -> Format（保持原输出维度）_1/1  "Cast（数据类型转换）"
  Cast（数据类型转换）_539/1 -> Format（保持原输出维度）_3/1  "Cast（数据类型转换）"
  Cast（数据类型转换）_542/1 -> Format（保持原输出维度）_4/1  "Cast（数据类型转换）"
  Cast（数据类型转换）_536/1 -> Format（保持原输出维度）_2/1  "Cast（数据类型转换）"
  Format（保持原输出维度）_5/1 -> Bleed（放气反馈）_546/1
  Format（保持原输出维度）_3/1 -> Aux（副阀反馈）_540/1
  Format（保持原输出维度）_4/1 -> Valve（阀使能反馈）_543/1
  Format（保持原输出维度）_2/1 -> Main（主阀反馈）_537/1

== system turbo_controller/BoardInput_输入换算与协议解析/In08_FRAM（复位数据转交） ==
  note: 把FRAM恢复结果交到旧控制接口
      |
      | 输入是FRAM事务模块给出的一次性恢复通知和20字节恢复内容。本层保持原有接口的数据类型和维度，
      | 将两者转交为ResetFlag与ResetInfo，供根层20 ms控制交接。
      |
      | 这里不读取SPI，不重算CRC，也不从20字节中提取油泵给定或转速。SPI收发、双区校验和一次性通知
      | 在FRAM_复位恢复事务中完成；字段解码在COMMRead_ISM/ECUReset_Information_Read完成。
      |
      | 通知表示“现在允许考虑恢复这份内容”，数据数组表示“要恢复什么”，二者不能分开理解。数组有
      | 数值本身不代表恢复已启用。
      |
      | 当前COMMRead_ISM内部把实际恢复解码许可接到false常量，外部ResetFlag被终止。因此本模块具备通
      | 知和内容的转交，但现有后级连线没有真正采用这一路恢复许可。
  Flag（复位恢复通知）_547 : Inport  OutDataTypeStr=uint8
  Info（复位恢复内容）_548 : Inport  Port=2  OutDataTypeStr=uint8
  Cast（数据类型转换）_549 : DataTypeConversion  OutDataTypeStr=uint8  RndMeth=Round
  Cast（数据类型转换）_551 : DataTypeConversion  OutDataTypeStr=uint8  RndMeth=Round
  Constant（常量）_553 : Constant  Value=zeros(50,1)  OutDataTypeStr=uint8
  Format（保持原输出维度）_1 : Reshape
  Vector1D（保持原一维向量接口）_2 : Reshape
  Vector1D（保持原一维向量接口）_3 : Reshape
  Flag（转交恢复通知）_550 : Outport
  Info（转交二十字节恢复内容）_552 : Outport  Port=2
  Setting（原预留五十字节装订接口）_554 : Outport  Port=3
  wires:
  Vector1D（保持原一维向量接口）_2/1 -> Info（转交二十字节恢复内容）_552/1
  Info（复位恢复内容）_548/1 -> Cast（数据类型转换）_551/1  "Info（复位恢复内容）"
  Cast（数据类型转换）_551/1 -> Vector1D（保持原一维向量接口）_2/1  "Cast（数据类型转换）"
  Vector1D（保持原一维向量接口）_3/1 -> Setting（原预留五十字节装订接口）_554/1
  Constant（常量）_553/1 -> Vector1D（保持原一维向量接口）_3/1  "Constant（常量）"
  Format（保持原输出维度）_1/1 -> Flag（转交恢复通知）_550/1
  Flag（复位恢复通知）_547/1 -> Cast（数据类型转换）_549/1  "Flag（复位恢复通知）"
  Cast（数据类型转换）_549/1 -> Format（保持原输出维度）_1/1  "Cast（数据类型转换）"

== system turbo_controller/BoardOutput_串口封装与阀门时序/Out01_Pump（泵反馈解析与滤波） ==
  note: 油泵反馈怎样解析并平滑
      |
      | 这里接收USART2的油泵回包字节和有效数量。逐字节寻找AA55帧头，收齐22字节并通过CRC16后，才取
      | 第6、7字节，按高字节在前合成原始泵速：
      | 本次原始反馈 = 高字节 × 256 + 低字节。
      |
      | 有效新帧到来时，不立即把输出完全跳到新值，而按原模型加权：
      | 本次泵速 = 0.875 × 上次泵速 + 0.125 × 本次原始反馈。
      | 例如上次输出800、新反馈1000，本次输出825。后续继续收到1000时再逐步接近，减少反馈跳动。
      |
      | 没有新有效帧时保持旧输出。这里的0.125更新只随有效回包发生，不能当成每毫秒都用相同数据再滤
      | 波一次。
      |
      | 该反馈交给Out03_Telemetry，拆成高低字节填入上位机回传帧；它不决定油泵的给定值。输入侧In03_
      | Pump是另一条预留校验路径，不能与本模块混淆。
  Rx（串口接收字节）_555 : Inport  OutDataTypeStr=uint8
  Count（有效字节数）_556 : Inport  Port=2  OutDataTypeStr=uint32
  Format（保持原输出维度）_1 : Reshape
  Receive（逐字节组帧与保持有效结果）_680 : Subsystem  Description=|
      | 实际油泵反馈接收流程：按1→2→3→4阅读
      | 
      | 第一步只遍历本批有效字节，最多处理64项；第二步识别AA55、收齐22字节，并保存尚未收完的半帧；第三步确认本字节刚收齐且CRC通过；第四步换算数值并保存最近有效结果。
      | 
      | Loop在一次调用内逐字节重复这些步骤，不是每一步各等1 ms。接收数组的Index每批重新遍历，收帧Position可以跨批保留，两者不是同一个位置。
      | 
      | 有效帧第6、7字节合成泵反馈，按0.875旧值+0.125新值更新；没有新帧时不重复滤波。
      | 
      | 本次将原有处理块按职责封装，保留原协议、初始化、数据类型、校验和循环行为。各步骤内部可看输入、公式和例子。
  Speed（反馈转速）_681 : Outport
  wires:
  Count（有效字节数）_556/1 -> Receive（逐字节组帧与保持有效结果）_680/2(Count（本次有效字节数）_558)  "Count（有效字节数）"
  Rx（串口接收字节）_555/1 -> Receive（逐字节组帧与保持有效结果）_680/1(Rx（本次接收字节）_557)  "Rx（串口接收字节）"
  Format（保持原输出维度）_1/1 -> Speed（反馈转速）_681/1
  Receive（逐字节组帧与保持有效结果）_680/1(Speed（当前有效反馈）_679) -> Format（保持原输出维度）_1/1  "Receive（逐字节组帧与保持有效结果）"

== system turbo_controller/BoardOutput_串口封装与阀门时序/Out02_Timing（阀门与点火时序） ==
  note: 阀门周期和点火请求怎样变成引脚电平
      |
      | 输入来自执行控制总线，本层每1 ms运行。先取出主阀、副阀的Enable、Cycle、Open，以及点火与引
      | 气请求。Cycle/Open是周期内的计数，不是已经生成的电平。
      |
      | 主阀和副阀分别交给MainValve、AuxValve。两者按2 ms节拍推进周期位置，位置小于Open时逻辑开启
      | ；使能为零或Cycle为零时关闭。例：Cycle=30、Open=15，对应约60 ms周期、前30 ms开启。
      | Ignition把非零点火请求变成10 ms循环中的前9 ms接通、最后1 ms断开。
      |
      | 然后才做电路极性映射：主阀、副阀、引气和点火的实际驱动支路按本页取反/比较变成低有效电平。
      | 软件On=true表示要求开启，不意味着GPIO一定为高。
      |
      | PortE顺序为副阀、主阀、引气的低有效电平，对应根层PE7、PE8、PE10。
      | PortD顺序为主阀使能高有效镜像、主阀逻辑开启镜像、点火低有效电平，对应PD11、PD12、PD13。
      |
      | 输出只整理为三项数组交给官方Digital Port Write。模式选择已经在CLM完成，本层按收到的要求排
      | 时序。
  Control（执行控制总线）_682 : Inport  OutDataTypeStr=Bus: EngineControl_Out
  AuxLow（副阀低有效输出）_765 : Logic  Operator=NOT  Inputs=1  IconShape=distinctive  AllPortsSameDT=off  OutDataTypeStr=boolean
  AuxValve（副阀周期与开度）_747 : Subsystem  Description=|
      | 副阀怎样按周期形成开启区间
      | 
      | 本模块收到使能Enable、周期计数Cycle、开启计数Open，以及父级给出的偶数毫秒节拍Even。它输出的是逻辑开启状态On，父级随后才按低有效电路把它取反成引脚电平。
      | 
      | 先检查Enable是否非零、Cycle是否非零，两者都成立才允许运行。对Cycle为零的情况，SafeCycle提供1作为取余用的安全分母，但运行许可仍为假，所以不会因为避免除零而误开阀。
      | 
      | 内部Phase记住周期位置，在2 ms节拍内按先归一化、后推进的分支更新。位置到周期末尾通过取余回到起点；位置小于Open时On为真，其余区间为假。
      | 
      | 例如Cycle=30、Open=15，约每60 ms重复一次，其中约30 ms开启；Open=0则没有开启区间，Open不小于周期时允许区间覆盖整个周期。这里的15是15个2 ms计数，不是15 ms。
      | 
      | 禁止使能时按关闭支路处理，不能仅看历史Phase猜测当前输出。位置跨1 ms调用保存，是周期波形成立所必需的状态。
  BleedLow（放气低有效输出）_768 : RelationalOperator  Operator===  OutDataTypeStr=boolean  RndMeth=Simplest  InputSameDT=off
  Cast（数据类型转换）_685 : DataTypeConversion  OutDataTypeStr=double  RndMeth=Round
  Constant（常量）_686 : Constant  Value=2  OutDataTypeStr=double
  Constant（常量）_688 : Constant  Value=0  OutDataTypeStr=double
  Constant（常量）_690 : Constant  OutDataTypeStr=uint32
  Constant（常量）_767 : Constant  Value=0  OutDataTypeStr=uint8
  Constant（常量）_770 : Constant  Value=0  OutDataTypeStr=uint8
  EnableHigh（阀使能高有效）_771 : RelationalOperator  Operator=~=  OutDataTypeStr=boolean  RndMeth=Simplest  InputSameDT=off
  Even（每两毫秒更新阀门相位）_689 : RelationalOperator  Operator===  OutDataTypeStr=boolean  RndMeth=Simplest  InputSameDT=off
  Fields（取主阀副阀点火与放气给定）_683 : BusSelector  OutputSignals=EValve_Enable,EValve_Cycle,EValve_Open,Eblast_Enable,Eblast_Cycle,Eblast_Open,SWO_Firework,SWO_BleedAir
  FireLow（点火低有效输出）_772 : Logic  Operator=NOT  Inputs=1  IconShape=distinctive  AllPortsSameDT=off  OutDataTypeStr=boolean
  Ignition（点火九毫秒开一毫秒关）_764 : Subsystem  Description=|
      | 点火请求怎样形成九开一关的节奏
      | 
      | 输入Request是点火请求，非零表示允许点火；它不是已经产生的脉冲。内部Phase按每1 ms调用推进，在0～9之间循环：
      | 下一位置 = mod(当前位置 + 1,10)。
      | 
      | 当请求有效且当前位置小于9时，On=true；位置等于9时On=false。因此每10 ms中前9 ms接通、最后1 ms断开，周期约100 Hz，逻辑占空比90%。
      | 
      | 请求无效时，输出关闭并把位置清零。下一次请求到来从新周期起点开始，不继续沿用停火前的位置。
      | 输出On交父级FireLow取反，生成低有效点火引脚电平。所以本图“开启”为真与实际引脚为低是同一动作的两种表示。
      | 
      | uint8用于保存0～9的相位；这里先取余再存储，不依赖整数溢出制造周期。
  MainLow（主阀低有效输出）_766 : Logic  Operator=NOT  Inputs=1  IconShape=distinctive  AllPortsSameDT=off  OutDataTypeStr=boolean
  MainValve（主阀周期与开度）_719 : Subsystem  Description=|
      | 主阀怎样按周期形成开启区间
      | 
      | 本模块收到使能Enable、周期计数Cycle、开启计数Open，以及父级给出的偶数毫秒节拍Even。它输出的是逻辑开启状态On，父级随后才按低有效电路把它取反成引脚电平。
      | 
      | 先检查Enable是否非零、Cycle是否非零，两者都成立才允许运行。对Cycle为零的情况，SafeCycle提供1作为取余用的安全分母，但运行许可仍为假，所以不会因为避免除零而误开阀。
      | 
      | 内部Phase记住周期位置，在2 ms节拍内按先归一化、后推进的分支更新。位置到周期末尾通过取余回到起点；位置小于Open时On为真，其余区间为假。
      | 
      | 例如Cycle=30、Open=15，约每60 ms重复一次，其中约30 ms开启；Open=0则没有开启区间，Open不小于周期时允许区间覆盖整个周期。这里的15是15个2 ms计数，不是15 ms。
      | 
      | 禁止使能时按关闭支路处理，不能仅看历史Phase猜测当前输出。位置跨1 ms调用保存，是周期波形成立所必需的状态。
  Phase2（两毫秒节拍）_687 : Math  Operator=mod
  PortD（D口三路电平顺序）_773 : Mux  Inputs=3
  PortD（D口三路输出电平）_776 : Reshape  OutputDimensionality=Column vector (2-D)
  PortE（E口三路电平顺序）_769 : Mux  Inputs=3
  PortE（E口三路输出电平）_774 : Reshape  OutputDimensionality=Column vector (2-D)
  Store_uint32（按三十二位无符号数保存状态）_537151 : DataTypeConversion  Description=为反馈回路显式指定原程序的状态类型，保持原状态更新节拍。  OutDataTypeStr=uint32  RndMeth=Round
  TickNext（毫秒计数按原规则饱和）_691 : Sum  SaturateOnIntegerOverflow=on  OutDataTypeStr=Inherit: Same as first input
  Tick（从零开始的毫秒计数）_684 : UnitDelay  InitialCondition=uint32(0)  SampleTime=-1  HasFrameUpgradeWarning=on
  PortE（E口三路输出电平）_775 : Outport
  PortD（D口三路输出电平）_777 : Outport  Port=2
  wires:
  PortD（D口三路输出电平）_776/1 -> PortD（D口三路输出电平）_777/1  "PortD（D口三路输出电平）"
  PortD（D口三路电平顺序）_773/1 -> PortD（D口三路输出电平）_776/1  "PortD（D口三路电平顺序）"
  PortE（E口三路输出电平）_774/1 -> PortE（E口三路输出电平）_775/1  "PortE（E口三路输出电平）"
  PortE（E口三路电平顺序）_769/1 -> PortE（E口三路输出电平）_774/1  "PortE（E口三路电平顺序）"
  FireLow（点火低有效输出）_772/1 -> PortD（D口三路电平顺序）_773/3  "FireLow（点火低有效输出）"
  EnableHigh（阀使能高有效）_771/1 -> PortD（D口三路电平顺序）_773/1  "EnableHigh（阀使能高有效）"
  Ignition（点火九毫秒开一毫秒关）_764/1(On（本毫秒点火接通）_763) -> FireLow（点火低有效输出）_772/1  "Ignition（点火九毫秒开一毫秒关）"
  Constant（常量）_770/1 -> EnableHigh（阀使能高有效）_771/2  "Constant（常量）"
  BleedLow（放气低有效输出）_768/1 -> PortE（E口三路电平顺序）_769/3  "BleedLow（放气低有效输出）"
  MainLow（主阀低有效输出）_766/1 -> PortE（E口三路电平顺序）_769/2  "MainLow（主阀低有效输出）"
  AuxLow（副阀低有效输出）_765/1 -> PortE（E口三路电平顺序）_769/1  "AuxLow（副阀低有效输出）"
  Constant（常量）_767/1 -> BleedLow（放气低有效输出）_768/2  "Constant（常量）"
  Fields（取主阀副阀点火与放气给定）_683/8 -> BleedLow（放气低有效输出）_768/1  "<SWO_BleedAir>"
  MainValve（主阀周期与开度）_719/1(On（逻辑开启状态）_718) -> MainLow（主阀低有效输出）_766/1, PortD（D口三路电平顺序）_773/2  "MainValve（主阀周期与开度）"
  AuxValve（副阀周期与开度）_747/1(On（逻辑开启状态）_746) -> AuxLow（副阀低有效输出）_765/1  "AuxValve（副阀周期与开度）"
  Fields（取主阀副阀点火与放气给定）_683/7 -> Ignition（点火九毫秒开一毫秒关）_764/1(Request（点火请求）_748)  "<SWO_Firework>"
  Fields（取主阀副阀点火与放气给定）_683/6 -> AuxValve（副阀周期与开度）_747/3(Open（开启计数）_723)  "<Eblast_Open>"
  Fields（取主阀副阀点火与放气给定）_683/5 -> AuxValve（副阀周期与开度）_747/2(Cycle（周期计数）_721)  "<Eblast_Cycle>"
  Fields（取主阀副阀点火与放气给定）_683/4 -> AuxValve（副阀周期与开度）_747/1(Enable（阀门使能）_720)  "<Eblast_Enable>"
  Even（每两毫秒更新阀门相位）_689/1 -> MainValve（主阀周期与开度）_719/4(Even（本毫秒为偶数节拍）_697), AuxValve（副阀周期与开度）_747/4(Even（本毫秒为偶数节拍）_725)  "Even（每两毫秒更新阀门相位）"
  Fields（取主阀副阀点火与放气给定）_683/3 -> MainValve（主阀周期与开度）_719/3(Open（开启计数）_695)  "<EValve_Open>"
  Fields（取主阀副阀点火与放气给定）_683/2 -> MainValve（主阀周期与开度）_719/2(Cycle（周期计数）_693)  "<EValve_Cycle>"
  Fields（取主阀副阀点火与放气给定）_683/1 -> MainValve（主阀周期与开度）_719/1(Enable（阀门使能）_692), EnableHigh（阀使能高有效）_771/1  "<EValve_Enable>"
  Constant（常量）_688/1 -> Even（每两毫秒更新阀门相位）_689/2  "Constant（常量）"
  Phase2（两毫秒节拍）_687/1 -> Even（每两毫秒更新阀门相位）_689/1  "Phase2（两毫秒节拍）"
  Constant（常量）_686/1 -> Phase2（两毫秒节拍）_687/2  "Constant（常量）"
  Control（执行控制总线）_682/1 -> Fields（取主阀副阀点火与放气给定）_683/1  "Control（执行控制总线）"
  Store_uint32（按三十二位无符号数保存状态）_537151/1 -> Tick（从零开始的毫秒计数）_684/1
  Tick（从零开始的毫秒计数）_684/1 -> TickNext（毫秒计数按原规则饱和）_691/1, Cast（数据类型转换）_685/1  "Tick（从零开始的毫秒计数）"
  Cast（数据类型转换）_685/1 -> Phase2（两毫秒节拍）_687/1  "Cast（数据类型转换）"
  Constant（常量）_690/1 -> TickNext（毫秒计数按原规则饱和）_691/2  "Constant（常量）"
  TickNext（毫秒计数按原规则饱和）_691/1 -> Store_uint32（按三十二位无符号数保存状态）_537151/1  "TickNext（毫秒计数按原规则饱和）"

== system turbo_controller/BoardOutput_串口封装与阀门时序/Out03_Telemetry（上位机回传组帧） ==
  note: 把回传字段组成一帧上位机数据
      |
      | 上层Send总线是若干字段，不是可以直接发出的最终串口字节数组。本模块同时接收Out01_Pump解析出
      | 的实际泵速，并按Clock20ms的许可，每20 ms生成一次通信更新。
      |
      | FrameCounter在更新时推进0～255循环帧号；PumpBytes把平滑泵速取整为16位，再拆成高、低两字节
      | 。
      | Payload先按原协议映射字段，加入AA55及类型01头部，然后明确覆盖第23字节帧号、第27字节泵速高
      | 字节、第28字节泵速低字节。
      |
      | Checksum对这28字节计算累加和异或校验，并追加到末尾，形成30字节帧。发送长度与回传开关、更新
      | 节拍共同决定本周期是否交给UART4发送，非更新时不能把相同数组误当新帧不断发送。
      |
      | 外层Bus Creator3有29个字段，那是总线接口数量；这里的30是最终串口帧字节数，二者不应直接比较
      | 成“长度不一致”。实际硬件发送由根层UART4_发送协议帧完成。
  Send（回传与外设命令总线）_114 : Inport  OutDataTypeStr=Bus: SendData_Out
  Pump（滤波后的油泵转速）_115 : Inport  Port=2  OutDataTypeStr=single
  Seconds（当前秒数）_116 : Inport  Port=3  OutDataTypeStr=double
  Checksum（累加与异或校验）_211 : Subsystem  Description=|
      | 一段字节怎样得到累加和异或两种校验
      | 
      | 输入是一整段需要校验的字节。每帧开始，两路累积值都从0开始；For Iterator按顺序取出每个字节，同时更新两路结果。
      | 
      | 累加这一路只保留低8位：
      | 新累加值 = mod(旧累加值 + 当前字节,256)。
      | 例如三个字节为200、100、1，总和301，最后校验字节为45，不让普通uint8溢出替代明确的取余规则。
      | 
      | 异或这一路逐位计算：
      | 新异或值 = bitxor(旧异或值,当前字节)。
      | 相同比特异或得到0，不同比特得到1。它与“所有数相加”是两种不同检查。
      | 
      | 接收侧拿这两个结果和帧尾比较，发送侧把结果追加到帧尾。父级负责规定哪些字节参加计算；本模块不验证帧头，也不能替换电机/油泵协议使用的CRC16。
  Clock20ms（二十毫秒通信节拍）_126 : Subsystem  Description=|
      | 从秒数产生每二十毫秒一次的许可
      | 
      | 本模块收到当前模型时间Seconds。先乘1000换成毫秒，再对20取余，判断余数是否小于1：
      | 工作许可 = mod(Seconds×1000,20)<1。
      | 
      | 在父级1 ms离散调用下，约在0、20、40、60 ms等时刻为真，中间毫秒为假。用“小于1”表示当前1 ms时间格，避免把它理解成连续时间的一次精确相等判断。
      | 
      | 这只是一个布尔许可，不会让模型等待或暂停。转速选择用它决定何时更新Speed，回传组帧用它决定何时生成新帧；其他1 ms任务继续正常运行。
  Constant（常量）_213 : Constant  Value=zeros(30,1)  OutDataTypeStr=uint8
  Constant（常量）_218 : Constant  Value=30  OutDataTypeStr=uint16
  Constant（常量）_219 : Constant  Value=0  OutDataTypeStr=uint16
  Format（保持原输出维度）_2 : Reshape
  Frame20ms（其他毫秒输出零帧）_214 : Switch  Criteria=u2 ~= 0  SaturateOnIntegerOverflow=off  InputSameDT=off
  Frame30（追加两字节校验）_212 : Mux  Inputs=3
  FrameCounter（循环帧号）_138 : Subsystem  Description=|
      | 用循环帧号辨认相邻回传帧
      | 
      | 输入Tick表示本次是否到20 ms通信更新时刻。内部记忆块保存上一帧号，本模块在Tick有效时加1，达到字节上限后回到0；Tick无效时保持。
      | 
      | 更新规律可理解为下一帧号=mod(旧帧号+1,256)。例如旧值254，下一次255，再下一次0，而不是让uint8相加后出现未说明的溢出。
      | 
      | 帧号交给Payload，覆盖最终28字节内容中的第23项，帮助上位机观察帧的先后和是否漏接。它不是发动机状态、转速，也不是已经运行的秒数。
  Length（发送三十字节或不发送）_220 : Switch  Criteria=u2 ~= 0  SaturateOnIntegerOverflow=off  InputSameDT=off
  Payload（原字段映射与覆盖）_195 : Subsystem  Description=|
      | 每个回传字段怎样放进固定字节位置
      | 
      | 输入Send是上层原回传字段总线，Counter是本帧循环帧号，High/Low是实际泵速的两个字节。本模块先按协议顺序取字段并转成uint8，最前面加入十六进制AA、55、01三项，构成28字节待校验内容。
      | 
      | 接着执行三次明确覆盖：第23字节改成本帧帧号；第27字节改成实际泵速高字节；第28字节改成实际泵速低字节。
      | 这三次Assignment发生在原字段拼接之后，因此对应位置最终以覆盖值为准，不能只读Original28的拼接顺序判断串口内容。
      | 
      | 例如平滑泵速1000会以高3、低232进入第27/28字节；帧号从255回0时只改变第23项。SendEnabled另外判断原回传开关是否非零，它是发送许可，不占一个新的帧数据位置。
      | 
      | 输出28字节交Checksum计算两项校验，父级再追加为30字节最终帧。本模块不直接启动UART。
  PumpBytes（泵速转高低字节）_152 : Subsystem  Description=|
      | 把泵速拆成高字节和低字节
      | 
      | 输入来自Out01_Pump的平滑反馈泵速，可能仍有小数。先按本页既有取整和uint16转换规则得到16位值U，再拆成两个可放进协议帧的字节：
      | 高字节 = floor(U/256)；
      | 低字节 = bitand(U,255)。
      | 
      | 例如U=1000，高字节为3、低字节为232，因为3×256+232=1000。上位机必须把两个字节按同样顺序合起来，不能把232单独当成完整泵速。
      | 
      | High和Low交给Payload，分别覆盖第27和28字节。这里只有数据编码，不再低通滤波，也没有修改油泵给定命令。
  SendNow（节拍与回传开关同时有效）_217 : Logic  IconShape=distinctive  AllPortsSameDT=off  OutDataTypeStr=boolean
  Tx4（上位机三十字节回传帧）_215 : Reshape  OutputDimensionality=Column vector (2-D)
  Tx4（上位机三十字节回传帧）_216 : Outport
  Length4（回传发送长度）_221 : Outport  Port=2
  wires:
  Constant（常量）_219/1 -> Length（发送三十字节或不发送）_220/3  "Constant（常量）"
  SendNow（节拍与回传开关同时有效）_217/1 -> Length（发送三十字节或不发送）_220/2  "SendNow（节拍与回传开关同时有效）"
  Constant（常量）_218/1 -> Length（发送三十字节或不发送）_220/1  "Constant（常量）"
  Payload（原字段映射与覆盖）_195/2(Enabled（上位机回传开关有效）_194) -> SendNow（节拍与回传开关同时有效）_217/2  "Payload（原字段映射与覆盖）"
  Tx4（上位机三十字节回传帧）_215/1 -> Tx4（上位机三十字节回传帧）_216/1  "Tx4（上位机三十字节回传帧）"
  Frame20ms（其他毫秒输出零帧）_214/1 -> Tx4（上位机三十字节回传帧）_215/1  "Frame20ms（其他毫秒输出零帧）"
  Constant（常量）_213/1 -> Frame20ms（其他毫秒输出零帧）_214/3  "Constant（常量）"
  Frame30（追加两字节校验）_212/1 -> Frame20ms（其他毫秒输出零帧）_214/1  "Frame30（追加两字节校验）"
  Checksum（累加与异或校验）_211/2(Xor8（八位异或结果）_210) -> Frame30（追加两字节校验）_212/3  "Checksum（累加与异或校验）"
  Checksum（累加与异或校验）_211/1(Sum8（八位累加结果）_209) -> Frame30（追加两字节校验）_212/2  "Checksum（累加与异或校验）"
  Payload（原字段映射与覆盖）_195/1(Payload（不含校验的二十八字节）_191) -> Checksum（累加与异或校验）_211/1(Bytes（待校验字节）_196), Frame30（追加两字节校验）_212/1  "Payload（原字段映射与覆盖）"
  PumpBytes（泵速转高低字节）_152/2(Low（泵速低字节）_151) -> Payload（原字段映射与覆盖）_195/4(Low（泵速低字节）_156)  "PumpBytes（泵速转高低字节）"
  PumpBytes（泵速转高低字节）_152/1(High（泵速高字节）_150) -> Payload（原字段映射与覆盖）_195/3(High（泵速高字节）_155)  "PumpBytes（泵速转高低字节）"
  FrameCounter（循环帧号）_138/1(Counter（当前帧使用的帧号）_137) -> Payload（原字段映射与覆盖）_195/2(Counter（本帧帧号）_154)  "FrameCounter（循环帧号）"
  Send（回传与外设命令总线）_114/1 -> Payload（原字段映射与覆盖）_195/1(Send（原回传字段总线）_153)  "Send（回传与外设命令总线）"
  Pump（滤波后的油泵转速）_115/1 -> PumpBytes（泵速转高低字节）_152/1(Pump（滤波后的油泵转速）_139)  "Pump（滤波后的油泵转速）"
  Clock20ms（二十毫秒通信节拍）_126/1(Every20ms（二十毫秒更新许可）_125) -> FrameCounter（循环帧号）_138/1(Control（二十毫秒更新许可）_127), SendNow（节拍与回传开关同时有效）_217/1, Frame20ms（其他毫秒输出零帧）_214/2  "Clock20ms（二十毫秒通信节拍）"
  Seconds（当前秒数）_116/1 -> Clock20ms（二十毫秒通信节拍）_126/1(Seconds（当前秒数）_117)  "Seconds（当前秒数）"
  Format（保持原输出维度）_2/1 -> Length4（回传发送长度）_221/1
  Length（发送三十字节或不发送）_220/1 -> Format（保持原输出维度）_2/1  "Length（发送三十字节或不发送）"
